simulink model "ESVW"  (R2022a)
settings: Solver=FixedStepAuto  StartTime=0.0  StopTime=10.0  RelTol=1e-3
settings Model: Creator=student  LastModifiedBy=student
settings OptimizationCC: DefaultParameterBehavior=Inlined  EnhancedBackFolding=on  PassReuseOutputArgsAs=Individual arguments  ZeroExternalMemoryAtStartup=off  ZeroInternalMemoryAtStartup=off  OptimizeBlockOrder=speed  DifferentSizesBufferReuse=on  OptimizationCustomize=off  EfficientTunableParamExpr=on
settings DebuggingCC: ParameterTunabilityLossMsg=error
settings HardwareCC: TargetBitPerPointer=64  TargetBitPerSizeT=64  TargetBitPerPtrDiffT=64  TargetLongLongMode=on  TargetIntDivRoundTo=Zero  TargetEndianess=LittleEndian  TargetWordSize=64  TargetHWDeviceType=MATLAB Host  ProdEqTarget=off
settings SFSimCC: MATLABDynamicMemAlloc=off
settings RTWCC: SystemTargetFile=ert.tlc  TemplateMakefile=ert_default_tmf
settings CodeAppCC: ForceParamTrailComments=on  IgnoreCustomStorageClasses=off  OperatorAnnotations=on  SimulinkDataObjDesc=on  SFDataObjDesc=on  InsertBlockDesc=on
settings ERTTargetCC: TargetLangStandard=C99 (ISO)  GenerateSampleERTMain=on  InlinedParameterPlacement=NonHierarchical  ERTCustomFileTemplate=example_file_process.tlc

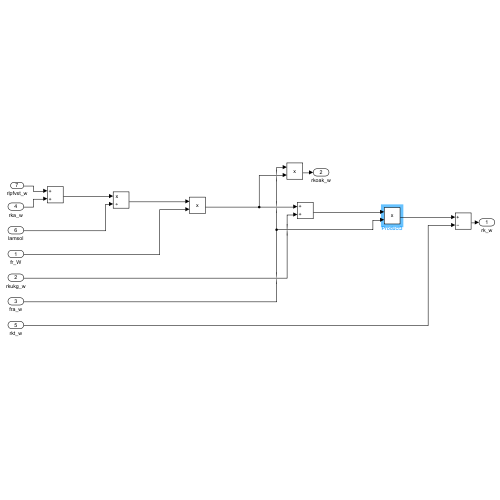
[thumbnail: Simulink's stored preview of the top-level diagram]
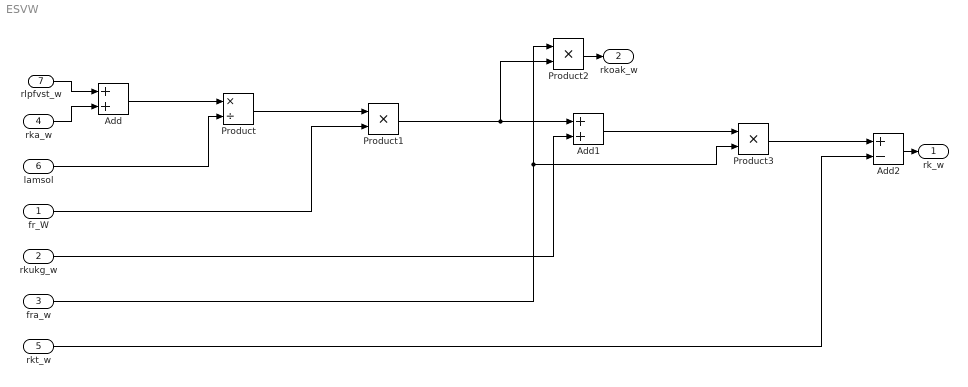
== system ESVW ==
  fr_W : Inport  OutMin=[0]  OutMax=[1.99997]  OutDataTypeStr=fixdt(0,16,1/32768,0)
  rkukg_w : Inport  Port=2  OutMin=[0]  OutMax=[3071.95]  OutDataTypeStr=fixdt(0,16,3/64,0)
  fra_w : Inport  Port=3  OutMin=[0]  OutMax=[1.99997]  OutDataTypeStr=fixdt(0,16,1/32768,0)
  rka_w : Inport  Port=4  OutMin=[0]  OutMax=[3071.95]  OutDataTypeStr=fixdt(0,16,3/64,0)
  rkt_w : Inport  Port=5  OutMin=[0]  OutMax=[3071.95]  OutDataTypeStr=fixdt(0,16,3/64,0)
  lamsol : Inport  Port=6  OutMin=[0]  OutMax=[15.999]  OutDataTypeStr=fixdt(0,16,1/4096,0)
  rlpfvst_w : Inport  Port=7  OutMin=[0]  OutMax=[3071.95]  OutDataTypeStr=fixdt(0,16,3/64,0)
  Add : Sum  AccumDataTypeStr=uint16  SaturateOnIntegerOverflow=on
  Add1 : Sum  OutDataTypeStr=uint16  SaturateOnIntegerOverflow=on
  Add2 : Sum  Inputs=+-  OutMin=[0]  OutMax=[3071.95]  OutDataTypeStr=fixdt(0,16,3/64,0)  SaturateOnIntegerOverflow=on
  Product : Product  Inputs=*/  OutDataTypeStr=uint16  SaturateOnIntegerOverflow=on
  Product1 : Product  OutDataTypeStr=uint16  SaturateOnIntegerOverflow=on
  Product2 : Product  OutMin=[0]  OutMax=[3071.95]  OutDataTypeStr=fixdt(0,16,3/64,0)  SaturateOnIntegerOverflow=on
  Product3 : Product  OutDataTypeStr=uint16  SaturateOnIntegerOverflow=on
  rk_w : Outport  OutMin=[0]  OutMax=[3071.95]  OutDataTypeStr=fixdt(0,16,3/64,0)
  rkoak_w : Outport  Port=2  OutMin=[0]  OutMax=[3071.95]  OutDataTypeStr=fixdt(0,16,3/64,0)
  wires:
  rkt_w/1 -> Add2/2
  Product2/1 -> rkoak_w/1
  Add2/1 -> rk_w/1
  Product3/1 -> Add2/1
  rkukg_w/1 -> Add1/2
  Product1/1 -> Add1/1, Product2/2
  Product/1 -> Product1/1
  rka_w/1 -> Add/2
  fr_W/1 -> Product1/2
  rlpfvst_w/1 -> Add/1
  fra_w/1 -> Product3/2, Product2/1
  lamsol/1 -> Product/2
  Add/1 -> Product/1
  Add1/1 -> Product3/1
